simulink model "IntegratedBehaviorModule"  (R2026a)
settings: Solver=VariableStepAuto  StopTime=inf
StartFcn:
  | clf
  | rng(1,"twister");
undefined symbols (not defined in the file): dem, fixedControllerParams, goalPose, initialTranslationTruck, mapSize, nlobjTracking, pathBus_struct, startPose, tuneableControllerParamsCpp, tuneableTerrainAwareParams, worldGridLoc, worldMat, worldRes
libraries: helperlib x5, simulink x4, robotmobilelib x1, offroadsim3dlib x1, sim3dlib x1
settings Model: Creator=cstabile  LastModifiedBy=merwinmendoza
settings DebuggingCC: IntegerOverflowMsg=none
settings SFSimCC: SFSimEcho=off  SimTargetLang=C++
settings RTWCC: SystemTargetFile=ert.tlc  Toolchain=Colcon Tools  Description=Embedded Coder
settings ERTTargetCC: RootIOFormat=Structure reference  DynamicArrayContainerType=coder::array

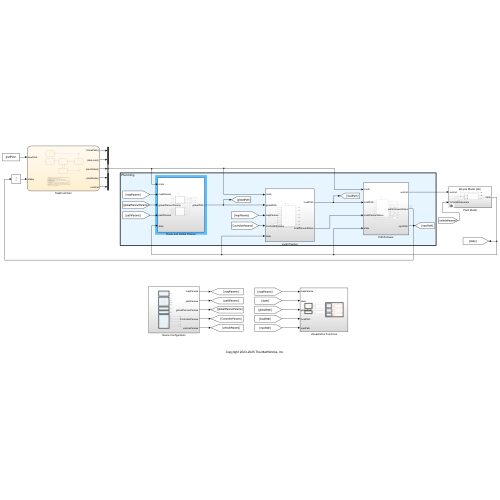
[thumbnail: Simulink's stored preview of the top-level diagram]
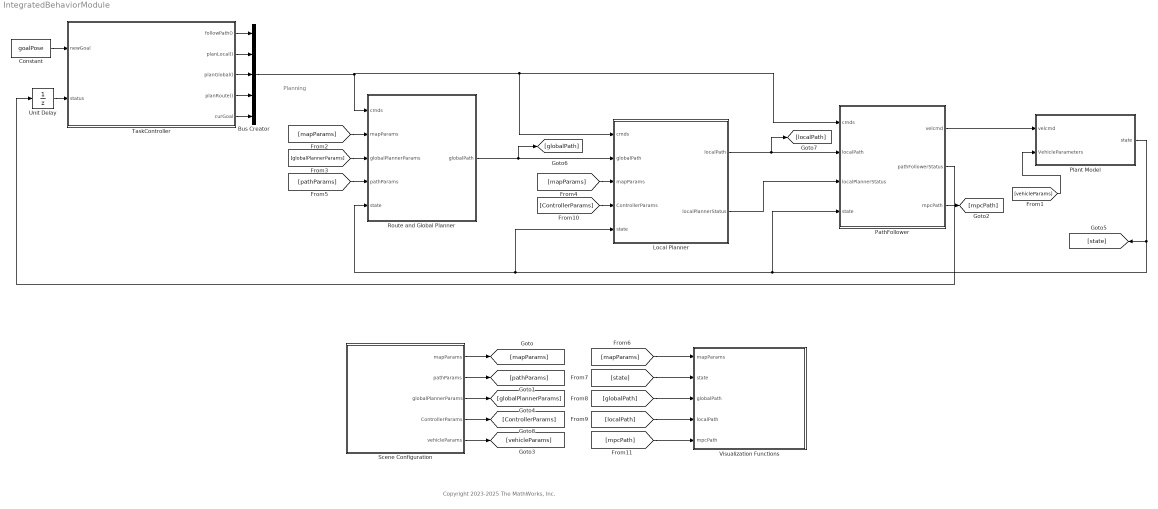
== system IntegratedBehaviorModule ==
  note: Planning
  note: Copyright 2023-2025 The MathWorks, Inc.
  Bus Creator : BusCreator  Inputs=5
  Constant : Constant  Value=goalPose
  Local Planner : Subsystem
  PathFollower : Subsystem
  Plant Model : Subsystem  Variant=on  VariantControlMode=label  VariantControl=Environemnt  LabelModeActiveChoice=Simple
  Route and Global Planner : Subsystem
  Scene Configuration : Subsystem
  TaskController : Stateflow chart  TreatAsAtomicUnit=on
      settings: PortSchema="{\"entries\":[{\"content\":{\"sides\":[{\"content\":{\"connectorIds\":[\"In1\",\"In2\"]},\"type\":\"ConnectorPlacement.EquallySpacedRectSide\",\"uuid\":\"cbfa7659-89a5-4e0b-94c8-c3ff629b6c07\"},{\"content\":{\"connectorIds\":[\"Out2\",\"Out3\",\"Out4\",\"Out5\",\"Out1\"],\"side\":\"RIGHT\"},\"type\":\"ConnectorPlacement.EquallySpacedRectSide\",\"uuid\":\"09a77d14-4924-404f-bc0a-d1cd3933e1ef\"},{\"content\":{\"side\":\"TOP\"},\"type\":\"ConnectorPlacement.EquallySpacedRectSide\",\"uuid\":\"bb1c4e19-123f-41f1-a220-47cc74084463\"},{\"content\":{\"side\":\"BOTTOM\"},\"type\":\"ConnectorPlacement.EquallySpacedRectSide\",\"uuid\":\"552a6ba0-446b-4106-9b79-f1f9bbf379fd\"}]},\"type\":\"ConnectorPlacement.EquallySpacedConnector\",\"uuid\":\"cd7ce687-884d-40d4-a1d1-e5ac9833bd00\"}],\"packageUris\":[\"http://schema.mathworks.com/mf0/Connector/R2020b\"],\"version\":\"1.0\"}"
  Unit Delay : UnitDelay  SampleTime=-1
  Visualization Functions : Subsystem
  wires:
  TaskController/2(followPath()) -> Bus Creator/1
  TaskController/3(planLocal()) -> Bus Creator/2
  TaskController/4(planGlobal()) -> Bus Creator/3
  TaskController/5(planRoute()) -> Bus Creator/4
  Scene Configuration/1(mapParams) -> [mapParams]
  Scene Configuration/2(pathParams) -> [pathParams]
  Scene Configuration/3(globalPlannerParams) -> [globalPlannerParams]
  Plant Model/1(state) -> PathFollower/4(state), Route and Global Planner/5(state), Local Planner/5(state), [state]
  PathFollower/1(velcmd) -> Plant Model/1(velcmd)
  [vehicleParams] -> Plant Model/2(VehicleParameters)
  Scene Configuration/4(ControllerParams) -> [ControllerParams]
  Scene Configuration/5(vehicleParams) -> [vehicleParams]
  Bus Creator/1 -> PathFollower/1(cmds), Local Planner/1(cmds), Route and Global Planner/1(cmds)
  [mapParams] -> Route and Global Planner/2(mapParams)
  [globalPlannerParams] -> Route and Global Planner/3(globalPlannerParams)
  [pathParams] -> Route and Global Planner/4(pathParams)
  [mapParams] -> Local Planner/3(mapParams)
  Route and Global Planner/1(globalPath) -> [globalPath], Local Planner/2(globalPath)
  [ControllerParams] -> Local Planner/4(ControllerParams)
  Local Planner/1(localPath) -> [localPath], PathFollower/2(localPath)
  Local Planner/2(localPlannerStatus) -> PathFollower/3(localPlannerStatus)
  Unit Delay/1 -> TaskController/2(status)
  PathFollower/2(pathFollowerStatus) -> Unit Delay/1
  [mapParams] -> Visualization Functions/1(mapParams)
  [state] -> Visualization Functions/2(state)
  [globalPath] -> Visualization Functions/3(globalPath)
  [localPath] -> Visualization Functions/4(localPath)
  Constant/1 -> TaskController/1(newGoal)
  PathFollower/3(mpcPath) -> [mpcPath]
  [mpcPath] -> Visualization Functions/5(mpcPath)
  TaskController/1(curGoal) -> Bus Creator/5

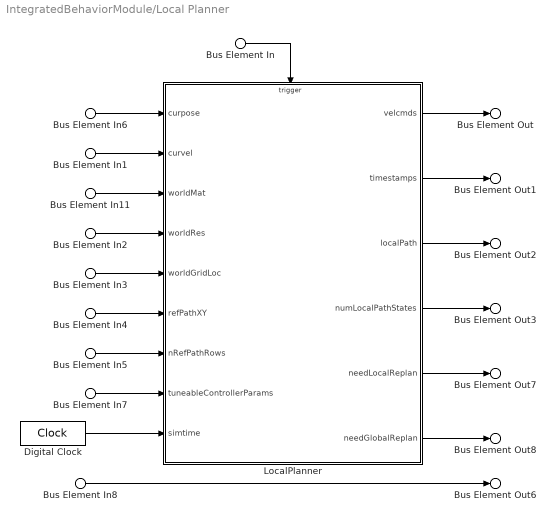
== system IntegratedBehaviorModule/Local Planner ==
  Bus Element In : Inport  PortName=cmds  Element=planLocal
  Bus Element In4 : Inport  Port=2  PortName=globalPath  Element=path
  Bus Element In5 : Inport  Port=2  PortName=globalPath  Element=numStates
  Bus Element In8 : Inport  Port=2  PortName=globalPath  Element=finalPose
  Bus Element In11 : Inport  Port=3  PortName=mapParams  Element=worldMat
  Bus Element In2 : Inport  Port=3  PortName=mapParams  Element=worldRes
  Bus Element In3 : Inport  Port=3  PortName=mapParams  Element=worldGridLoc
  Bus Element In7 : Inport  Port=4  PortName=ControllerParams  Element=allParams
  Bus Element In6 : Inport  Port=5  PortName=state  Element=pose
  Bus Element In1 : Inport  Port=5  PortName=state  Element=velocity
  Digital Clock : DigitalClock  SampleTime=nlobjTracking.Ts
  LocalPlanner : Subsystem  Variant=on  VariantControlMode=label  VariantControl=LocalPlanner  LabelModeActiveChoice=LocalPlannerMPPI
  Bus Element Out : Outport  PortName=localPath  Element=velcmds
  Bus Element Out1 : Outport  PortName=localPath  Element=timestamps
  Bus Element Out2 : Outport  PortName=localPath  Element=path
  Bus Element Out3 : Outport  PortName=localPath  Element=numStates
  Bus Element Out6 : Outport  PortName=localPath  Element=globalPathEndPose
  Bus Element Out7 : Outport  Port=2  PortName=localPlannerStatus  Element=needLocalReplan
  Bus Element Out8 : Outport  Port=2  PortName=localPlannerStatus  Element=needGlobalReplan
  wires:
  Bus Element In/1 -> LocalPlanner/Trigger
  Bus Element In6/1 -> LocalPlanner/1(curpose)
  Bus Element In1/1 -> LocalPlanner/2(curvel)
  Bus Element In11/1 -> LocalPlanner/3(worldMat)
  Bus Element In2/1 -> LocalPlanner/4(worldRes)
  Bus Element In3/1 -> LocalPlanner/5(worldGridLoc)
  Bus Element In4/1 -> LocalPlanner/6(refPathXY)
  Bus Element In5/1 -> LocalPlanner/7(nRefPathRows)
  Bus Element In7/1 -> LocalPlanner/8(tuneableControllerParams)
  Digital Clock/1 -> LocalPlanner/9(simtime)
  LocalPlanner/1(velcmds) -> Bus Element Out/1
  LocalPlanner/2(timestamps) -> Bus Element Out1/1
  LocalPlanner/3(localPath) -> Bus Element Out2/1
  LocalPlanner/4(numLocalPathStates) -> Bus Element Out3/1
  LocalPlanner/5(needLocalReplan) -> Bus Element Out7/1
  LocalPlanner/6(needGlobalReplan) -> Bus Element Out8/1
  Bus Element In8/1 -> Bus Element Out6/1

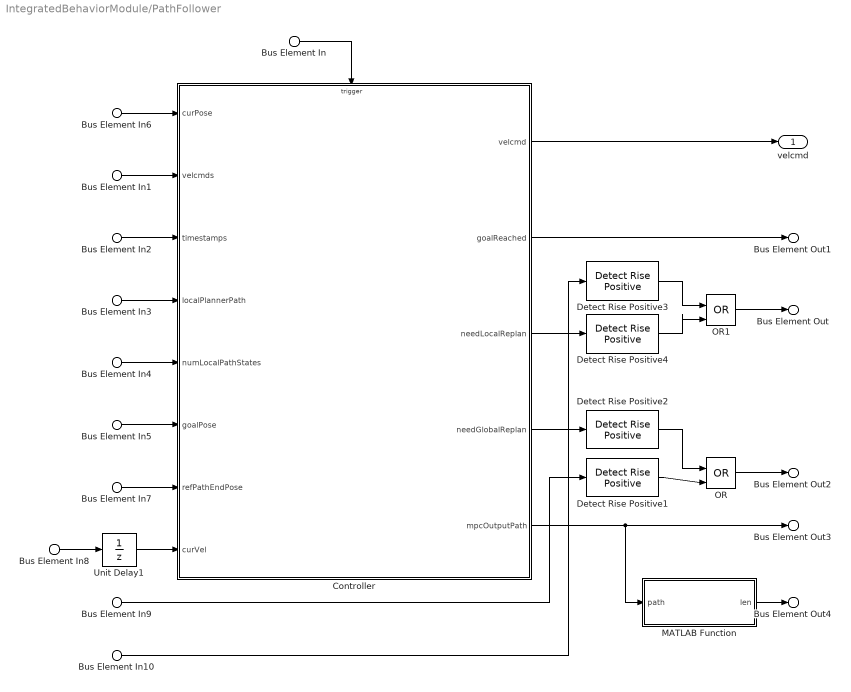
== system IntegratedBehaviorModule/PathFollower ==
  Bus Element In : Inport  PortName=cmds  Element=followPath
  Bus Element In5 : Inport  PortName=cmds  Element=curGoal
  Bus Element In1 : Inport  Port=2  PortName=localPath  Element=velcmds
  Bus Element In2 : Inport  Port=2  PortName=localPath  Element=timestamps
  Bus Element In3 : Inport  Port=2  PortName=localPath  Element=path
  Bus Element In4 : Inport  Port=2  PortName=localPath  Element=numStates
  Bus Element In7 : Inport  Port=2  PortName=localPath  Element=globalPathEndPose
  Bus Element In9 : Inport  Port=3  PortName=localPlannerStatus  Element=needGlobalReplan
  Bus Element In10 : Inport  Port=3  PortName=localPlannerStatus  Element=needLocalReplan
  Bus Element In6 : Inport  Port=4  PortName=state  Element=pose
  Bus Element In8 : Inport  Port=4  PortName=state  Element=velocity
  Controller : Subsystem  Variant=on  VariantControlMode=label  VariantControl=Controller  LabelModeActiveChoice=Local Planner MPC Cascade
  Detect Rise Positive{1..4} (4 alike) : simulink/Logic and Bit Operations/Detect Rise Positive  vinit=0  OutDataTypeStr=boolean
  MATLAB Function : MATLAB Function  TreatAsAtomicUnit=on
  OR : Logic  Operator=OR  IconShape=distinctive  AllPortsSameDT=off  OutDataTypeStr=boolean
  OR1 : Logic  Operator=OR  IconShape=distinctive  AllPortsSameDT=off  OutDataTypeStr=boolean
  Unit Delay1 : UnitDelay  SampleTime=-1
  velcmd : Outport
  Bus Element Out : Outport  Port=2  PortName=pathFollowerStatus  Element=needLocalReplan
  Bus Element Out2 : Outport  Port=2  PortName=pathFollowerStatus  Element=needGlobalReplan
  Bus Element Out1 : Outport  Port=2  PortName=pathFollowerStatus  Element=goalReached
  Bus Element Out3 : Outport  Port=3  PortName=mpcPath  Element=path
  Bus Element Out4 : Outport  Port=3  PortName=mpcPath  Element=numStates
  wires:
  Controller/1(velcmd) -> velcmd/1
  Controller/2(goalReached) -> Bus Element Out1/1
  Controller/4(needGlobalReplan) -> Detect Rise Positive2/1
  Detect Rise Positive2/1 -> OR/1
  Bus Element In7/1 -> Controller/7(refPathEndPose)
  Bus Element In8/1 -> Unit Delay1/1
  Unit Delay1/1 -> Controller/8(curVel)
  Controller/3(needLocalReplan) -> Detect Rise Positive4/1
  Bus Element In6/1 -> Controller/1(curPose)
  Bus Element In1/1 -> Controller/2(velcmds)
  Bus Element In2/1 -> Controller/3(timestamps)
  Bus Element In3/1 -> Controller/4(localPlannerPath)
  Bus Element In4/1 -> Controller/5(numLocalPathStates)
  Bus Element In5/1 -> Controller/6(goalPose)
  Bus Element In9/1 -> Detect Rise Positive1/1
  Detect Rise Positive1/1 -> OR/2
  OR/1 -> Bus Element Out2/1
  Bus Element In10/1 -> Detect Rise Positive3/1
  Detect Rise Positive3/1 -> OR1/1
  Detect Rise Positive4/1 -> OR1/2
  OR1/1 -> Bus Element Out/1
  Bus Element In/1 -> Controller/Trigger
  Controller/5(mpcOutputPath) -> MATLAB Function/1(path), Bus Element Out3/1
  MATLAB Function/1(len) -> Bus Element Out4/1

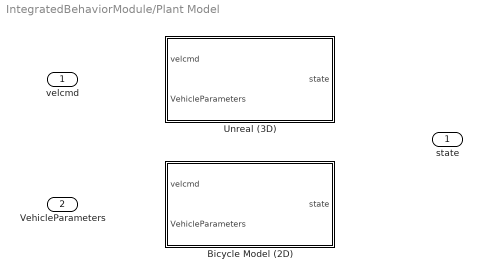
== system IntegratedBehaviorModule/Plant Model ==
  velcmd : Inport
  VehicleParameters : Inport  Port=2
  Bicycle Model (2D) : Subsystem  VariantControl=Simple
  Unreal (3D) : Subsystem  VariantControl=Unreal
  state : Outport

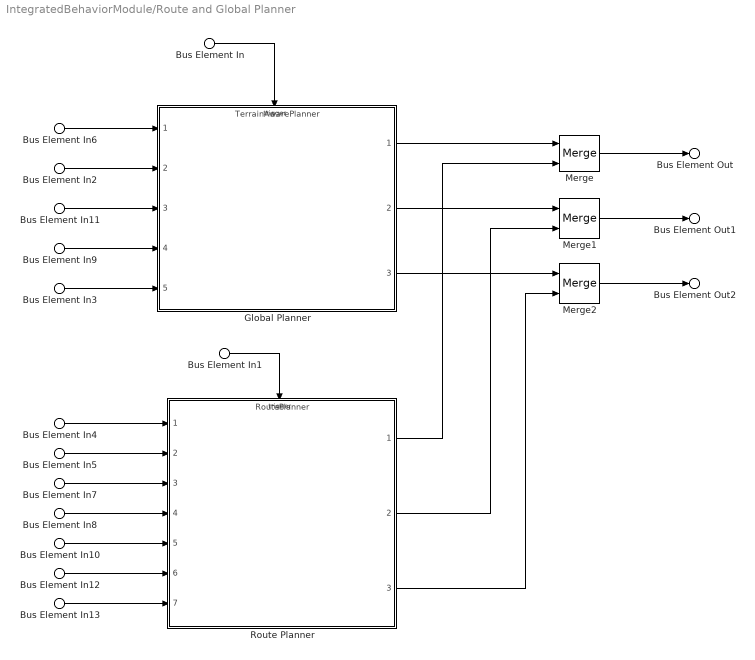
== system IntegratedBehaviorModule/Route and Global Planner ==
  Bus Element In : Inport  PortName=cmds  Element=planGlobal
  Bus Element In1 : Inport  PortName=cmds  Element=planRoute
  Bus Element In2 : Inport  PortName=cmds  Element=curGoal
  Bus Element In7 : Inport  PortName=cmds  Element=curGoal
  Bus Element In9 : Inport  Port=2  PortName=mapParams  Element=worldGridLoc
  Bus Element In10 : Inport  Port=2  PortName=mapParams  Element=worldGridLoc
  Bus Element In11 : Inport  Port=2  PortName=mapParams  Element=dem
  Bus Element In8 : Inport  Port=2  PortName=mapParams  Element=worldMat
  Bus Element In12 : Inport  Port=2  PortName=mapParams  Element=worldRes
  Bus Element In3 : Inport  Port=3  PortName=globalPlannerParams  Element=allParams
  Bus Element In13 : Inport  Port=3  PortName=globalPlannerParams  Element=allParams.MinTurningRadius
  Bus Element In4 : Inport  Port=4  PortName=pathParams  Element=pathBus
  Bus Element In6 : Inport  Port=5  PortName=state  Element=pose
  Bus Element In5 : Inport  Port=5  PortName=state  Element=pose
  Global Planner : ModelReference  ModelNameDialog=TerrainAwarePlanner.slx  SimulationMode=Normal  ModelReferenceVersion=5.0  TriggerPortName=Trigger  TriggerPortTriggerType=function-call  TriggerPortStatesWhenEnabling=held
  Merge : Merge
  Merge1 : Merge
  Merge2 : Merge
  Route Planner : ModelReference  ModelNameDialog=RoutePlanner.slx  SimulationMode=Normal  ModelReferenceVersion=3.2  TriggerPortName=Trigger  TriggerPortTriggerType=function-call  TriggerPortStatesWhenEnabling=held
  Bus Element Out : Outport  PortName=globalPath  Element=path
  Bus Element Out1 : Outport  PortName=globalPath  Element=numStates
  Bus Element Out2 : Outport  PortName=globalPath  Element=finalPose
  wires:
  Bus Element In12/1 -> Route Planner/6
  Bus Element In13/1 -> Route Planner/7
  Bus Element In/1 -> Global Planner/Trigger
  Global Planner/1 -> Merge/1
  Global Planner/2 -> Merge1/1
  Global Planner/3 -> Merge2/1
  Bus Element In1/1 -> Route Planner/Trigger
  Bus Element In3/1 -> Global Planner/5
  Bus Element In2/1 -> Global Planner/2
  Bus Element In6/1 -> Global Planner/1
  Bus Element In11/1 -> Global Planner/3
  Bus Element In9/1 -> Global Planner/4
  Bus Element In4/1 -> Route Planner/1
  Bus Element In5/1 -> Route Planner/2
  Bus Element In7/1 -> Route Planner/3
  Bus Element In8/1 -> Route Planner/4
  Bus Element In10/1 -> Route Planner/5
  Route Planner/1 -> Merge/2
  Route Planner/2 -> Merge1/2
  Route Planner/3 -> Merge2/2
  Merge/1 -> Bus Element Out/1
  Merge1/1 -> Bus Element Out1/1
  Merge2/1 -> Bus Element Out2/1

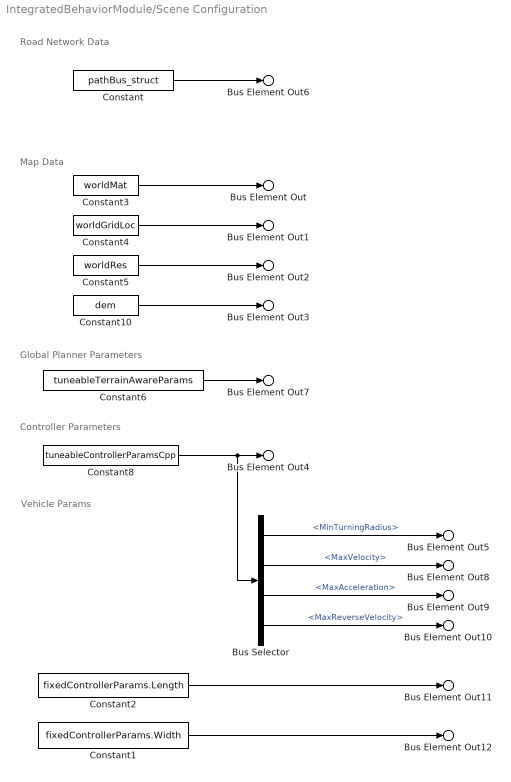
== system IntegratedBehaviorModule/Scene Configuration ==
  note: Vehicle Params
  note: Map Data
  note: Road Network Data
  note: Global Planner Parameters
  note: Controller Parameters
  Bus Selector : BusSelector  OutputSignals=MinTurningRadius,MaxVelocity,MaxAcceleration,MaxReverseVelocity
  Constant : Constant  Value=pathBus_struct  OutDataTypeStr=Bus: pathList_fixed_bus
  Constant1 : Constant  Value=fixedControllerParams.Width  VectorParams1D=off
  Constant10 : Constant  Value=dem
  Constant2 : Constant  Value=fixedControllerParams.Length  VectorParams1D=off
  Constant3 : Constant  Value=worldMat
  Constant4 : Constant  Value=worldGridLoc
  Constant5 : Constant  Value=worldRes
  Constant6 : Constant  Value=tuneableTerrainAwareParams  OutDataTypeStr=Bus: fsp_tunable_bus
  Constant8 : Constant  Value=tuneableControllerParamsCpp  OutDataTypeStr=Bus:controller_bus
  Bus Element Out : Outport  PortName=mapParams  Element=worldMat
  Bus Element Out1 : Outport  PortName=mapParams  Element=worldGridLoc
  Bus Element Out2 : Outport  PortName=mapParams  Element=worldRes
  Bus Element Out3 : Outport  PortName=mapParams  Element=dem
  Bus Element Out6 : Outport  Port=2  PortName=pathParams  Element=pathBus
  Bus Element Out7 : Outport  Port=3  PortName=globalPlannerParams  Element=allParams
  Bus Element Out4 : Outport  Port=4  PortName=ControllerParams  Element=allParams
  Bus Element Out5 : Outport  Port=5  PortName=vehicleParams  Element=MinTurningRadius
  Bus Element Out8 : Outport  Port=5  PortName=vehicleParams  Element=MaxVelocity
  Bus Element Out9 : Outport  Port=5  PortName=vehicleParams  Element=MaxAcceleration
  Bus Element Out10 : Outport  Port=5  PortName=vehicleParams  Element=MaxReverseVelocity
  Bus Element Out11 : Outport  Port=5  PortName=vehicleParams  Element=Length
  Bus Element Out12 : Outport  Port=5  PortName=vehicleParams  Element=Width
  wires:
  Constant10/1 -> Bus Element Out3/1
  Constant/1 -> Bus Element Out6/1
  Constant8/1 -> Bus Selector/1, Bus Element Out4/1
  Constant5/1 -> Bus Element Out2/1
  Constant6/1 -> Bus Element Out7/1
  Constant4/1 -> Bus Element Out1/1
  Constant3/1 -> Bus Element Out/1
  Bus Selector/4 -> Bus Element Out10/1  "<MaxReverseVelocity>"
  Bus Selector/2 -> Bus Element Out8/1  "<MaxVelocity>"
  Constant2/1 -> Bus Element Out11/1
  Bus Selector/3 -> Bus Element Out9/1  "<MaxAcceleration>"
  Bus Selector/1 -> Bus Element Out5/1  "<MinTurningRadius>"
  Constant1/1 -> Bus Element Out12/1

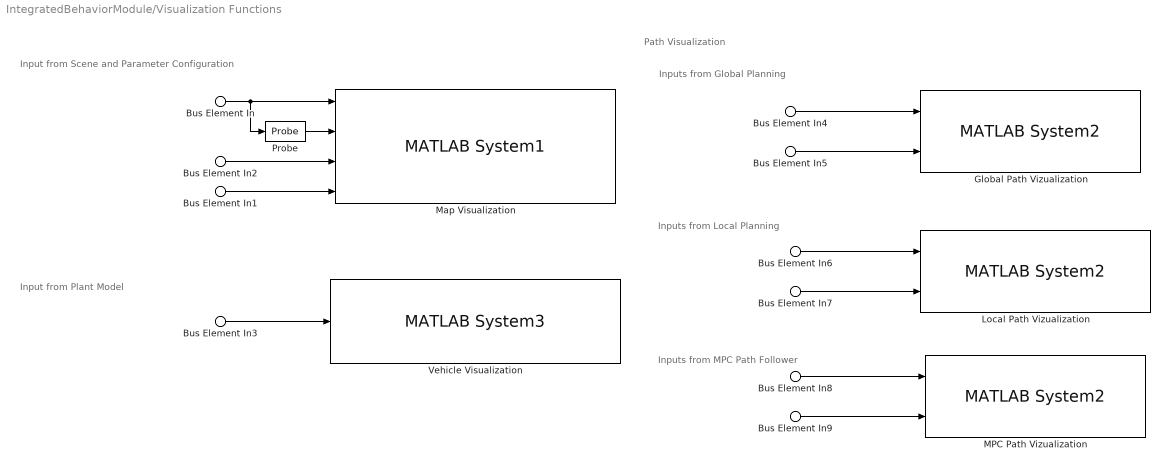
== system IntegratedBehaviorModule/Visualization Functions ==
  note: Input from Scene and Parameter Configuration
  note: Inputs from Global Planning
  note: Input from Plant Model
  note: Inputs from Local Planning
  note: Inputs from MPC Path Follower
  note: Path Visualization
  Bus Element In : Inport  PortName=mapParams  Element=worldMat
  Bus Element In1 : Inport  PortName=mapParams  Element=worldGridLoc
  Bus Element In2 : Inport  PortName=mapParams  Element=worldRes
  Bus Element In3 : Inport  Port=2  PortName=state  Element=pose
  Bus Element In4 : Inport  Port=3  PortName=globalPath  Element=path
  Bus Element In5 : Inport  Port=3  PortName=globalPath  Element=numStates
  Bus Element In6 : Inport  Port=4  PortName=localPath  Element=path
  Bus Element In7 : Inport  Port=4  PortName=localPath  Element=numStates
  Bus Element In8 : Inport  Port=5  PortName=mpcPath  Element=path
  Bus Element In9 : Inport  Port=5  PortName=mpcPath  Element=numStates
  Global Path Vizualization : helperlib/MATLAB System2  VisualizationParameters={'Color','#D95319','LineWidth',3}  PlotType=Line  Legend=Global Path  DisplayVisual=on  SimulateUsing=Interpreted execution
  Local Path Vizualization : helperlib/MATLAB System2  VisualizationParameters={'c:','LineWidth',3}  PlotType=Line  Legend=Local Path  DisplayVisual=on  SimulateUsing=Interpreted execution
  MPC Path Vizualization : helperlib/MATLAB System2  VisualizationParameters={'k:','LineWidth',3}  PlotType=Line  Legend=MPC Output Path  DisplayVisual=on  SimulateUsing=Interpreted execution
  Map Visualization : helperlib/MATLAB System1  MapType=Bin  DisplayVisual=on  SimulateUsing=Interpreted execution
  Probe : Probe  ProbeWidth=off  ProbeSampleTime=off  ProbeComplexSignal=off  ProbeSignalDimensions=on
  Vehicle Visualization : helperlib/MATLAB System3  NumCircles=3  Length=fixedControllerParams.Length  Width=fixedControllerParams.Width  DisplayVisual=on  SimulateUsing=Interpreted execution
  wires:
  Bus Element In/1 -> Map Visualization/1, Probe/1
  Bus Element In1/1 -> Map Visualization/4
  Bus Element In5/1 -> Global Path Vizualization/2
  Bus Element In2/1 -> Map Visualization/3
  Bus Element In3/1 -> Vehicle Visualization/1
  Probe/1 -> Map Visualization/2
  Bus Element In4/1 -> Global Path Vizualization/1
  Bus Element In6/1 -> Local Path Vizualization/1
  Bus Element In7/1 -> Local Path Vizualization/2
  Bus Element In8/1 -> MPC Path Vizualization/1
  Bus Element In9/1 -> MPC Path Vizualization/2

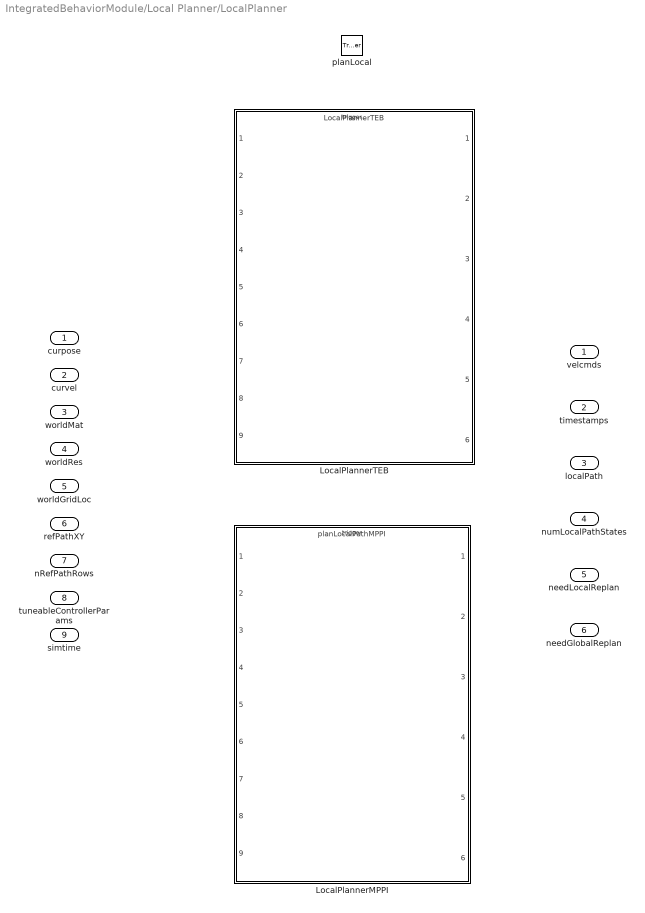
== system IntegratedBehaviorModule/Local Planner/LocalPlanner ==
  curpose : Inport
  curvel : Inport  Port=2
  worldMat : Inport  Port=3
  worldRes : Inport  Port=4
  worldGridLoc : Inport  Port=5
  refPathXY : Inport  Port=6
  nRefPathRows : Inport  Port=7
  tuneableControllerParams : Inport  Port=8
  simtime : Inport  Port=9
  planLocal : TriggerPort  TriggerType=function-call  VariantControl=(inherit)
  LocalPlannerMPPI : ModelReference  ModelNameDialog=planLocalPathMPPI.slx  SimulationMode=Normal  VariantControl=LocalPlannerMPPI  ModelReferenceVersion=6.0  TriggerPortName=planLocal  TriggerPortTriggerType=function-call  TriggerPortStatesWhenEnabling=held
  LocalPlannerTEB : ModelReference  ModelNameDialog=LocalPlannerTEB.slx  SimulationMode=Normal  VariantControl=LocalPlannerTEB  ModelReferenceVersion=6.0  TriggerPortName=planLocal  TriggerPortTriggerType=function-call  TriggerPortStatesWhenEnabling=held
  velcmds : Outport
  timestamps : Outport  Port=2
  localPath : Outport  Port=3
  numLocalPathStates : Outport  Port=4
  needLocalReplan : Outport  Port=5  OutDataTypeStr=boolean
  needGlobalReplan : Outport  Port=6  OutDataTypeStr=boolean

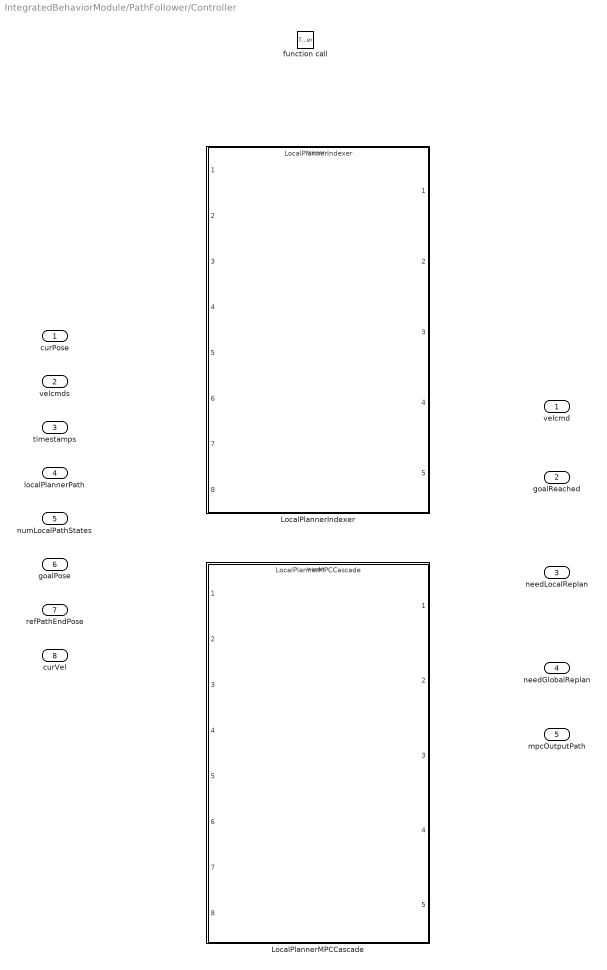
== system IntegratedBehaviorModule/PathFollower/Controller ==
  curPose : Inport
  velcmds : Inport  Port=2
  timestamps : Inport  Port=3
  localPlannerPath : Inport  Port=4
  numLocalPathStates : Inport  Port=5
  goalPose : Inport  Port=6
  refPathEndPose : Inport  Port=7
  curVel : Inport  Port=8
  function call : TriggerPort  TriggerType=function-call  VariantControl=(inherit)  PortDimensions=1
  LocalPlannerIndexer : ModelReference  ModelNameDialog=LocalPlannerIndexer  SimulationMode=Normal  VariantControl=Local Planner Indexer  ModelReferenceVersion=6.0  TriggerPortName=function call  TriggerPortTriggerType=function-call  TriggerPortStatesWhenEnabling=held
  LocalPlannerMPCCascade : ModelReference  ModelNameDialog=LocalPlannerMPCCascade  SimulationMode=Normal  VariantControl=Local Planner MPC Cascade  ModelReferenceVersion=6.0  TriggerPortName=function call  TriggerPortTriggerType=function-call  TriggerPortStatesWhenEnabling=held
  velcmd : Outport
  goalReached : Outport  Port=2
  needLocalReplan : Outport  Port=3
  needGlobalReplan : Outport  Port=4
  mpcOutputPath : Outport  Port=5

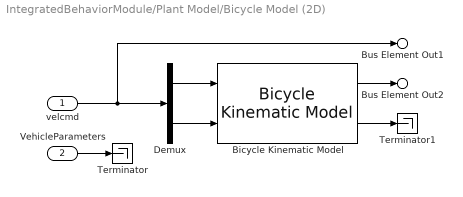
== system IntegratedBehaviorModule/Plant Model/Bicycle Model (2D) ==
  velcmd : Inport
  VehicleParameters : Inport  Port=2
  Bicycle Kinematic Model : robotmobilelib/Bicycle Kinematic Model  VehicleInputs=Vehicle Speed & Heading Angular Velocity  WheelBase=fixedControllerParams.Length  VehicleSpeedRange=[-inf inf]  MaxSteeringAngle=pi/4  InitialState=startPose  SimulateUsing=Interpreted execution
  Demux : Demux  Outputs=2
  Terminator : Terminator
  Terminator1 : Terminator
  Bus Element Out1 : Outport  PortName=state  Element=velocity
  Bus Element Out2 : Outport  PortName=state  Element=pose
  wires:
  VehicleParameters/1 -> Terminator/1
  velcmd/1 -> Bus Element Out1/1, Demux/1
  Demux/1 -> Bicycle Kinematic Model/1
  Bicycle Kinematic Model/2 -> Terminator1/1
  Demux/2 -> Bicycle Kinematic Model/2
  Bicycle Kinematic Model/1 -> Bus Element Out2/1

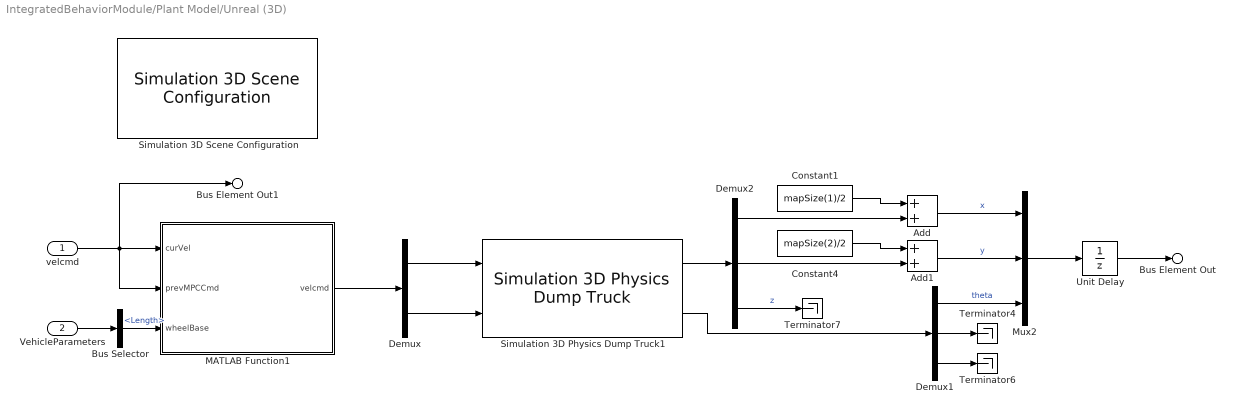
== system IntegratedBehaviorModule/Plant Model/Unreal (3D) ==
  velcmd : Inport  PortDimensions=[1 2]
  VehicleParameters : Inport  Port=2
  Add : Sum
  Add1 : Sum
  Bus Selector : BusSelector  OutputSignals=Length
  Constant1 : Constant  Value=mapSize(1)/2  VectorParams1D=off
  Constant4 : Constant  Value=mapSize(2)/2  VectorParams1D=off
  Demux : Demux  Outputs=2
  Demux1 : Demux  Outputs=3
  Demux2 : Demux  Outputs=3
  MATLAB Function1 : MATLAB Function  TreatAsAtomicUnit=on
  Mux2 : Mux  Inputs=3
  Simulation 3D Physics Dump Truck1 : offroadsim3dlib/Simulation 3D Physics Dump Truck  TruckType=Standard Dump Truck  TruckColor=Yellow  ActorName=SimulinkVehicle  InitTruckTrans=initialTranslationTruck  InitTruckRot=initialRotationTruck  InitTruckVel=0  InitTruckAccel=0  InitTruckBedAng=0  EnableCollisionVisualization=off  CollisionGeomColor=[0 1 0]  CollisionGeomTransp=0.1  EnbAccelInp=off  EnbFootBrakInp=off  EnbLifAngInp=off  EnbTruckTransOut=on  EnbTruckRotOut=on  EnbTruckVelOut=off  EnbTruckAngVelOut=off  EnbTruckBedTransOut=off  EnbTruckBedRotOut=off  EnbTruckBedAngOut=off  SampleTime=0.025  ActorType=SimulinkVehicle  ID=C  aMode=6  ActorTag=SimulinkVehicle  Mesh=DumpTruck
  Simulation 3D Scene Configuration : sim3dlib/Simulation 3D Scene Configuration  Priority=0  ProjectFormat=Default Scenes  SceneDesc=Offroad pit mining scene  ProjectName=Y:\41\apattass.BR2025ad.j2959407\matlab\toolbox\shared\sim3d_projects\automotive_project_windows\UE\WindowsNoEditor\VehicleSimulation.exe  ScenePath=/Game/Maps/HwStrght  EnableOpenDRIVE=off  vehTagList={'Custom';'Scene Origin';'SimulinkVehicle'}  vehTag=SimulinkVehicle  AttachedCameraRelativeTranslation=[0 0 0]  FreeCameraDefaultInitialTranslation=[-6, 0, 2]  AttachedCameraRelativeRotation=[0 0 0]  FreeCameraDefaultInitialRotation=[0, -15, 0]  ViewpointName=Custom  FreeCameraInitialTranslation=initialTranslationTruck([2 1 3]).*[1 -1 1] + [0 0 50]  ViewpointTranslation=[0 0 0]  FreeCameraInitialRotation=[0, 0, 0]  ViewpointRotation=[0 0 0]  OpVisEn=off  Ts=0.025  EnableWindow=on  EnableRemoteAccess=off  EnableWeather=off  SunAzimuth=90  SunAltitude=40.0  EnableGeospatialSun=off  Latitude=0  Longitude=0  Date=2023-01-01  Time=10:30:00  GeoTimeZone=-5.0  SunDaylightSaving=off  wind=1  clouds=10  EnableVolumetricClouds=off  CloudCoverage=0  CloudAltitude=6  fog=0  rain=0  RaindropsEffect=off  SnowDensity=0  EnableGeospatial=off  TilesetSource=Earth terrain  UseTrueOrigin=off  OriginHeight=200  OriginLatitude=40.744652  OriginLongitude=-73.988864  MapStyle=Aerial  AdditionalAssetIDs=[]  UseAdvancedSunSky=off  SolarTime=11  TimeZone=-5  Day=21  Month=9  Year=2022  UseDaylightSavingTime=on  DSTStartDay=10  DSTStartMonth=3  DSTEndDay=3  DSTEndMonth=11  DSTSwitchHour=2  sensorTag=MainCamera3  sensorId=3  sensorName=MainCamera3  mountLoc=Origin  offsetFlag=off  tmountOffset=[0, 0, 0]  rmountOffset=[0, 0, 0]  HorizontalResolution=1280  VerticalResolution=720  HorizontalFOV=60  mountPoint=[0 0 0]  mountOrientation=[0 0 0]  aMode=6  ID=3  GeoTrigger=Inactive  ViewNameList={'Custom'}  ViewTranslationList={'[-159 333 129.8783]'}  ViewRotationList={'[0 0 0]'}
      settings: LibrarySourceBlock=robotsim3dlib/Simulation 3D Scene Configuration
  Terminator4 : Terminator
  Terminator6 : Terminator
  Terminator7 : Terminator
  Unit Delay : UnitDelay  InitialCondition=startPose  SampleTime=-1
  Bus Element Out : Outport  PortName=state  Element=pose
  Bus Element Out1 : Outport  PortName=state  Element=velocity
  wires:
  Demux2/3 -> Terminator7/1  "z"
  Add/1 -> Mux2/1  "x"
  Demux1/2 -> Terminator4/1
  velcmd/1 -> Bus Element Out1/1, MATLAB Function1/2(prevMPCCmd), MATLAB Function1/1(curVel)
  Demux1/3 -> Terminator6/1
  Demux2/1 -> Add/2
  Constant1/1 -> Add/1
  Simulation 3D Physics Dump Truck1/1 -> Demux2/1
  Add1/1 -> Mux2/2  "y"
  Demux2/2 -> Add1/2
  Demux1/1 -> Mux2/3  "theta"
  Constant4/1 -> Add1/1
  VehicleParameters/1 -> Bus Selector/1
  Bus Selector/1 -> MATLAB Function1/3(wheelBase)  "<Length>"
  Demux/1 -> Simulation 3D Physics Dump Truck1/1
  Simulation 3D Physics Dump Truck1/2 -> Demux1/1
  Demux/2 -> Simulation 3D Physics Dump Truck1/2
  MATLAB Function1/1(velcmd) -> Demux/1
  Mux2/1 -> Unit Delay/1
  Unit Delay/1 -> Bus Element Out/1

== matlab function IntegratedBehaviorModule/PathFollower/MATLAB Function ==
  data: path input; len output
function len = findPathLength(path)

len = size(path,1);

== stateflow chart IntegratedBehaviorModule/TaskController ==
  state WaitingForTask
  state RoutePlanner
    entry:
    curGoal = newGoal;
    send(planRoute);
  state LocalPlanner
    entry:
    send(planLocal);
  state FollowingPath
    entry, during:
    send(followPath);
  state GlobalPlanner
    entry:
    send(planGlobal);
  note: Initial State : The model starts in the WaitingForTask state. Running the model changes the state to RoutePlanner.
      | RoutePlanner : Finds the path from start to goal, then moves to LocalPlanner state.
      | LocalPlanner : Determines the optimal trajectory and control, then moves to FollowingPath state.
      | FollowingPath : A controller generates smooth velocity commands to steer the vehicle along the optimal trajectory genereated by local planner.
      | GlobalPlanner : From LocalPlanner or FollowingPath, need for new global path move the state to GlobalPlanner.
  (junction 52) -> WaitingForTask
  FollowingPath -> (junction 52) [order 1] : [status.goalReached]
  WaitingForTask -> RoutePlanner : [hasChanged(newGoal)]
  RoutePlanner -> LocalPlanner
  LocalPlanner -> FollowingPath [order 2] : [~status.needLocalReplan]
  (default) -> RoutePlanner
  FollowingPath -> LocalPlanner [order 3] : [status.needLocalReplan || after(0.5, sec)]
  LocalPlanner -> GlobalPlanner [order 1] : [status.needGlobalReplan]
  GlobalPlanner -> LocalPlanner
  FollowingPath -> (junction 54) [order 2] : [status.needGlobalReplan]
  (junction 54) -> GlobalPlanner
  data: newGoal input double size=[1 3]; curGoal output size=[1 3]; status input Bus: pathStatusBus size=1
  events: followPath output FUNCTION_CALL_EVENT; planLocal output FUNCTION_CALL_EVENT; planGlobal output FUNCTION_CALL_EVENT; planRoute output FUNCTION_CALL_EVENT

== matlab function IntegratedBehaviorModule/Plant Model/Unreal (3D)/MATLAB Function1 ==
  data: curVel input; prevMPCCmd input; velcmd output; wheelBase input
function velcmd = vel2mpc(curVel,prevMPCCmd,wheelBase)
velcmd = curVel;
if velcmd(1) == 0
    % Use previous steering angle when velocity is 0
    velcmd(2) = prevMPCCmd(2);
else
    % Otherwise compute it from turn-rate
    velcmd(2) = atan(curVel(2)*wheelBase/velcmd(1));
end
velcmd = velcmd(:)';
velcmd = flip(velcmd);
